simulink model "simple_PID"  (R2024b)
settings: Solver=FixedStepAuto  StartTime=0.0  StopTime=15  FixedStep=1e-3  RelTol=1e-3
settings Model: Creator=kentliukx  LastModifiedBy=kentliukx

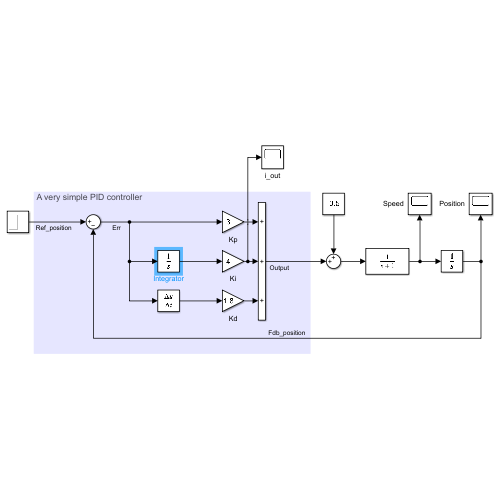
[thumbnail: Simulink's stored preview of the top-level diagram]
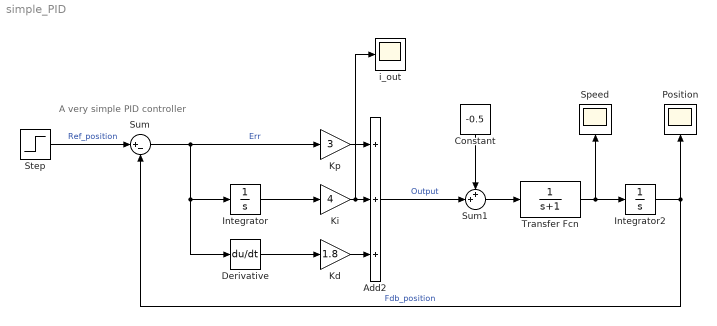
== system simple_PID ==
  note: A very simple PID controller
  Add2 : Sum  Inputs=+++
  Constant : Constant  Value=-0.5
  Derivative : Derivative
  Integrator : Integrator  UpperSaturationLimit=0.15  LowerSaturationLimit=-0.15
  Integrator2 : Integrator
  Kd : Gain  Gain=1.8
  Ki : Gain  Gain=4
  Kp : Gain  Gain=3
  Position : Scope
  Speed : Scope
  Step : Step  SampleTime=0
  Sum : Sum  Inputs=|+-
  Sum1 : Sum  Inputs=++|
  Transfer Fcn : TransferFcn  Denominator=[1 1]
  i_out : Scope
  wires:
  Ki/1 -> i_out/1, Add2/2
  Step/1 -> Sum/1  "Ref_position"
  Add2/1 -> Sum1/2  "Output"
  Kd/1 -> Add2/3
  Sum/1 -> Derivative/1, Integrator/1, Kp/1  "Err"
  Kp/1 -> Add2/1
  Transfer Fcn/1 -> Integrator2/1, Speed/1
  Integrator2/1 -> Position/1, Sum/2  "Fdb_position"
  Derivative/1 -> Kd/1
  Integrator/1 -> Ki/1
  Sum1/1 -> Transfer Fcn/1
  Constant/1 -> Sum1/1
